simulink model "VehicleModel_MVP_AI"  (R2026b)
settings: Solver=ode4  StopTime=90  FixedStep=0.005
values from neighbouring files (symbols this model uses):
  MVP = 0.02    [QuadInterfaces_AI.sldd]
libraries: uavalgslib x1
settings Model: DataDictionary=QuadInterfaces_AI.sldd  Creator=JonathanTee  LastModifiedBy=JonathanTee
settings ModelReferenceCC: ModelReferenceMinAlgLoopOccurrences=on

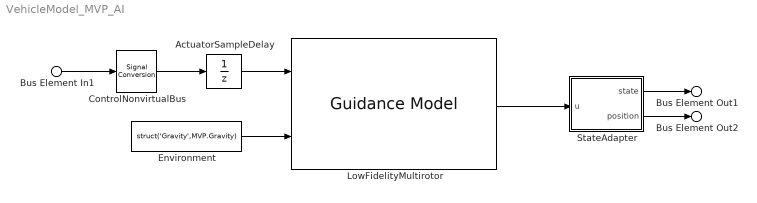
== system VehicleModel_MVP_AI ==
  Bus Element In1 : Inport  PortName=ControlOutputs
  ActuatorSampleDelay : UnitDelay  InitialCondition=struct('Roll',0,'Pitch',0,'YawRate',0,'Thrust',MVP.Mass*MVP.Gravity)  SampleTime=MVP.SampleTime
  ControlNonvirtualBus : SignalConversion  ConversionOutput=Nonvirtual bus  OverrideOpt=off
  Environment : Constant  Value=struct('Gravity',MVP.Gravity)  OutDataTypeStr=Bus: MVP_UAV_Environment
  LowFidelityMultirotor : uavalgslib/Guidance Model  ModelType=MultirotorGuidance  NumInstances=1  SpecifiedDataType=double  SimulateUsing=Interpreted execution  InitialWorldPositionMultirotor=MVP.InitialPosition  InitialWorldVelocityMultirotor=[0; 0; 0]  InitialEulerZYXMultirotor=[0; 0; 0]  InitialBodyAngularRateRPYMultirotor=[0; 0; 0]  InitialThrustMultirotor=MVP.Mass*MVP.Gravity  InitialNorthFixedWing=0  InitialEastFixedWing=0  InitialHeightFixedWing=0  InitialAirSpeedFixedWing=0  InitialHeadingAngleFixedWing=0  InitialFlightPathAngleFixedWing=0  InitialRollAngleFixedWing=0  InitialRollAngleRateFixedWing=0  PDRollMultirotor=MVP.AttitudePD  PDPitchMultirotor=MVP.AttitudePD  PYawRateMultirotor=MVP.YawRateGain  PThrustMultirotor=MVP.ThrustGain  MassMultirotor=MVP.Mass  PHeightFixedWing=3.9  PHeadingAngleFixedWing=3.9  PFlightPathAngleFixedWing=39  PDRollFixedWing=[3402.97, 116.67]  PAirSpeedFixedWing=1  FlightPathAngleLimitsFixedWing=[-pi/2, pi/2]  StateBusName='MVP_UAV_State'  ControlBusName='ControlOutputs_IF'  EnvironmentBusName='MVP_UAV_Environment'  DataType=double
  StateAdapter : MATLAB Function  TreatAsAtomicUnit=on
  Bus Element Out1 : Outport  PortName=VehicleState
  Bus Element Out2 : Outport  Port=2  PortName=Position
  wires:
  StateAdapter/2(position) -> Bus Element Out2/1
  StateAdapter/1(state) -> Bus Element Out1/1
  ActuatorSampleDelay/1 -> LowFidelityMultirotor/1
  LowFidelityMultirotor/1 -> StateAdapter/1(u)
  Environment/1 -> LowFidelityMultirotor/2
  Bus Element In1/1 -> ControlNonvirtualBus/1
  ControlNonvirtualBus/1 -> ActuatorSampleDelay/1

== matlab function VehicleModel_MVP_AI/StateAdapter ==
  data: u input Bus: MVP_UAV_State; state output Bus: VehicleState_IF; position output Bus: Position_IF
function [state,position]=adapt(u)
%#codegen
[state,position]=stage02_state_adapter(u);
end
